simulink model "LLC_simu"  (R2023a)
settings: Solver=VariableStepAuto  StartTime=0.0  StopTime=0.01  RelTol=1e-3
values from neighbouring files (symbols this model uses):
  Co = Co_s    [generate_agent_v2_cases.m]    (also in generate_aging_trajectory.m = co_ratio * Co_nominal; generate_dataset_2.m = co_samples; llc_agent_v2_cases.mat = [0.002046 0.00231 0.001936 0.00209 0.00198 0.002288 0.001892; llc_aging_trajectory.mat = [0.0022 0.002145 0.00209 0.002035 0.00198 0.001925 0.00187 0)
  Cr = Cr_s    [generate_agent_v2_cases.m]    (also in generate_aging_trajectory.m = Cr_nominal * ones(num_sequences, 1); generate_dataset_2.m = cr_samples; llc_agent_v2_cases.mat = [3.57e-08 3.36e-08 3.465e-08 4.55e-08 3.43e-08 3.605e-08 3.5; llc_aging_trajectory.mat = [3.5e-08 3.5e-08 3.5e-08 3.5e-08 3.5e-08 3.5e-08 3.5e-08 3.5)
  D = 45    [generate_agent_v2_cases.m]    (also in generate_aging_trajectory.m; generate_dataset_2.m; setparams.m)
  Lm = Lm_s    [generate_agent_v2_cases.m]    (also in generate_aging_trajectory.m = Lm_nominal * ones(num_sequences, 1); generate_dataset_2.m = lm_samples; llc_agent_v2_cases.mat = [0.00014162 0.0001022 0.00015184 0.00014892 0.00015038 0.000; llc_aging_trajectory.mat = [0.000146 0.000146 0.000146 0.000146 0.000146 0.000146 0.000)
  Lr = Lr_s    [generate_agent_v2_cases.m]    (also in generate_aging_trajectory.m = Lr_nominal * ones(num_sequences, 1); generate_dataset_2.m = lr_samples; llc_agent_v2_cases.mat = [9.49e-05 7.154e-05 7.519e-05 7.081e-05 7.446e-05 7.008e-05 ; llc_aging_trajectory.mat = [7.3e-05 7.3e-05 7.3e-05 7.3e-05 7.3e-05 7.3e-05 7.3e-05 7.3)
  Ro = rload_samples(k)    [generate_aging_trajectory.m]    (also in generate_dataset_2.m; setparams.m = 2)
  T = 1 / fs_k    [generate_agent_v2_cases.m]    (also in generate_aging_trajectory.m = 1.11111111111e-05; generate_dataset_2.m; setparams.m = 1.11111111111e-05)
  Vin = Vin_nominal    (= 311)    [generate_aging_trajectory.m]    (also in generate_dataset_2.m = vin_samples(k); setparams.m)
  Vpulse = 1    [generate_agent_v2_cases.m]    (also in generate_aging_trajectory.m; generate_dataset_2.m; setparams.m)
libraries: spsCurrentMeasurementLib x14, spsSeriesRLCBranchLib x5, spsVoltageMeasurementLib x5, spsDiodeLib x4, spsMosfetLib x4, spsLinearTransformerLib x1, spsDCVoltageSourceLib x1, spspowerguiLib x1
settings Model: Creator=22431  LastModifiedBy=22431
settings SimscapeCC: SimscapeNormalizeSystem=off

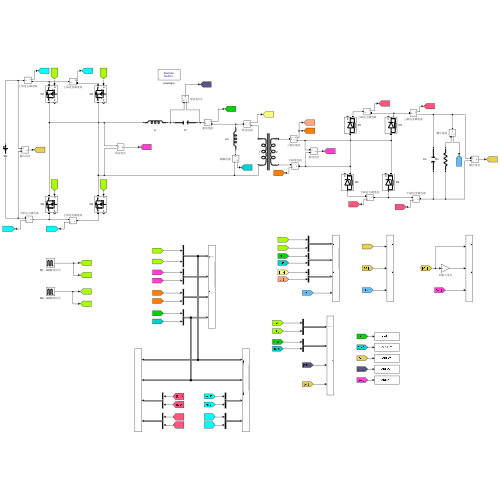
[thumbnail: Simulink's stored preview of the top-level diagram]
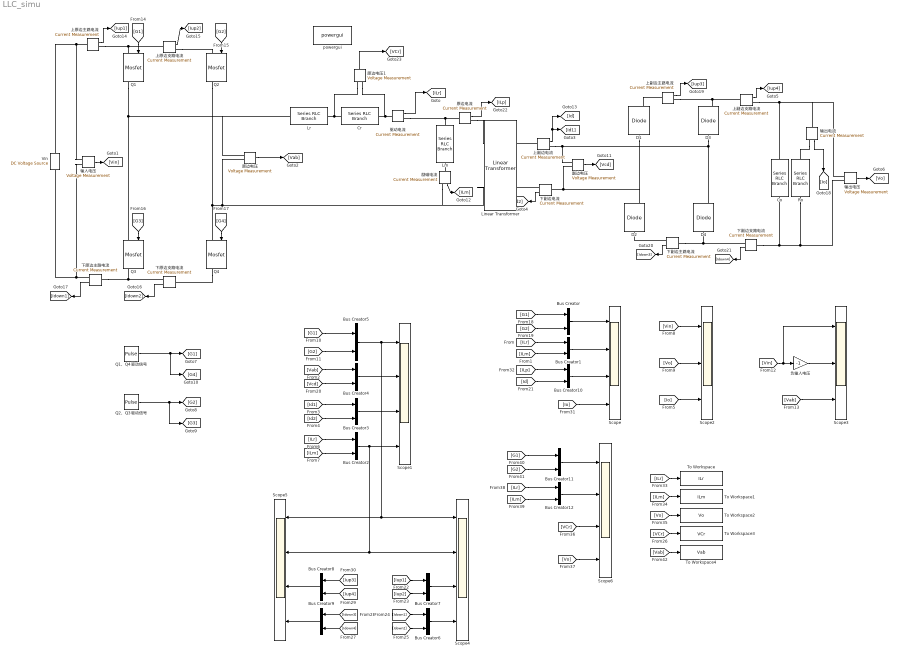
== system LLC_simu ==
  Bus Creator{,1..12} (13 alike) : BusCreator  Inputs=2
  Co : spsSeriesRLCBranchLib/Series RLC Branch  LConnTagsString=__new0  RConnTagsString=__new0  BranchType=C  Resistance=1  Inductance=1e-3  SetiL0=off  InitialCurrent=0  Capacitance=Co  Setx0=off  InitialVoltage=0  Measurements=None
  Cr : spsSeriesRLCBranchLib/Series RLC Branch  LConnTagsString=__new0  RConnTagsString=__new0  BranchType=C  Resistance=1  Inductance=1e-3  SetiL0=off  InitialCurrent=0  Capacitance=Cr  Setx0=off  InitialVoltage=0  Measurements=None
  D{1..4} (4 alike) : spsDiodeLib/Diode  Ron=0.001  Lon=0  Vf=0.8  IC=0  UseSnubber=0  Rs=500  Cs=250e-9  Measurements=on
  Linear Transformer : spsLinearTransformerLib/Linear Transformer  UNITS=SI  NominalPower=[ 250e6 100e3 ]  winding1=[6.5 0 0]  winding2=[1 0 0]  ThreeWindings=off  winding3=[1.5e+05 0 0]  RmLm=[1e6 inf]  Measurements=None  DataType=on
  Lm : spsSeriesRLCBranchLib/Series RLC Branch  LConnTagsString=__new0  RConnTagsString=__new0  BranchType=L  Resistance=1  Inductance=Lm  SetiL0=off  InitialCurrent=0  Capacitance=1e-6  Setx0=off  InitialVoltage=0  Measurements=None
  Lr : spsSeriesRLCBranchLib/Series RLC Branch  LConnTagsString=__new0  RConnTagsString=__new0  BranchType=L  Resistance=1  Inductance=Lr  SetiL0=off  InitialCurrent=0  Capacitance=1e-6  Setx0=off  InitialVoltage=0  Measurements=None
  Q{1..4} (4 alike) : spsMosfetLib/Mosfet  Ron=0.1  Lon=0  Rd=0.01  Vfd=0  IC=0  Rs=1e5  Cs=inf  Measurements=on
  Q1、Q4驱动信号 : DiscretePulseGenerator  PulseType=Time based  Amplitude=Vpulse  Period=T  PulseWidth=D
  Q2、Q3驱动信号 : DiscretePulseGenerator  PulseType=Time based  Amplitude=Vpulse  Period=T  PulseWidth=D  PhaseDelay=T/2
  Ro : spsSeriesRLCBranchLib/Series RLC Branch  LConnTagsString=__new0  RConnTagsString=__new0  BranchType=R  Resistance=Ro  Inductance=1e-3  SetiL0=off  InitialCurrent=0  Capacitance=1e-6  Setx0=off  InitialVoltage=0  Measurements=None
  Scope{,1,4..6} (5 alike) : Scope  NumInputPorts=4
  Scope2 : Scope  NumInputPorts=3
  Scope3 : Scope  NumInputPorts=3
  To Workspace : ToWorkspace  VariableName=ILr  SaveFormat=Timeseries  SampleTime=-1
  To Workspace1 : ToWorkspace  VariableName=ILm  SaveFormat=Timeseries  SampleTime=-1
  To Workspace2 : ToWorkspace  VariableName=Vo  SaveFormat=Timeseries  SampleTime=-1
  To Workspace3 : ToWorkspace  VariableName=VCr  SaveFormat=Timeseries  SampleTime=-1
  To Workspace4 : ToWorkspace  VariableName=Vab  SaveFormat=Timeseries  SampleTime=-1
  Vin : spsDCVoltageSourceLib/DC Voltage Source  Amplitude=Vin  Measurements=None
  powergui : spspowerguiLib/powergui  Priority=1  SimulationMode=Discrete  SampleTime=50e-10  frequency=60  Iterations=50  frequencyindice=0  Pbase=100e6  ErrMax=1e-4  UnitsV=kV  UnitsW=MW  buscounter=0  FunctionMessages=off  echomessages=off  EnableUseOfTLC=off  CurrentSourceSwitches=off  DisableSnubberDevices=off  DisableRonSwitches=off  DisableVfSwitches=off  DisplayEquations=off  AutomaticDiscreteSolvers=off  SolverType=Tustin/Backward Euler (TBE)  Interpol=off  ExternalGateDelay=off  methode=off  Ts=100  x0status=blocks  SPID=on  SwTol=0  HookPort=off  NonlinearTolerance=1e-4  nMaxIteration=100  ContinueOnMaxIteration=off  RestoreLinks=warning  ResistiveCurrentMeasurement=off  Frange=[0:2:500]  Ylog=off  Xlog=on  ShowGrid=off  save=off  variable=ZData  structure=0  ZoomFFT=off  StartTime=0.0  cycles=1  DisplayStyle=1  fundamental=60  FreqAxis=off  MaxFrequency=1000  frequencyindicesteady=1  RmsSteady=1  display=off
  上副边主路电流 : spsCurrentMeasurementLib/Current Measurement  PhasorSimulation=off  OutputType=Complex  PSBequivalent=0
  上副边支路电流 : spsCurrentMeasurementLib/Current Measurement  PhasorSimulation=off  OutputType=Complex  PSBequivalent=0
  上副边电流 : spsCurrentMeasurementLib/Current Measurement  PhasorSimulation=off  OutputType=Complex  PSBequivalent=0
  上原边主路电流 : spsCurrentMeasurementLib/Current Measurement  PhasorSimulation=off  OutputType=Complex  PSBequivalent=0
  上原边支路电流 : spsCurrentMeasurementLib/Current Measurement  PhasorSimulation=off  OutputType=Complex  PSBequivalent=0
  下副边主路电流 : spsCurrentMeasurementLib/Current Measurement  PhasorSimulation=off  OutputType=Complex  PSBequivalent=0
  下副边支路电流 : spsCurrentMeasurementLib/Current Measurement  PhasorSimulation=off  OutputType=Complex  PSBequivalent=0
  下副边电流 : spsCurrentMeasurementLib/Current Measurement  PhasorSimulation=off  OutputType=Complex  PSBequivalent=0
  下原边主路电流 : spsCurrentMeasurementLib/Current Measurement  PhasorSimulation=off  OutputType=Complex  PSBequivalent=0
  下原边支路电流 : spsCurrentMeasurementLib/Current Measurement  PhasorSimulation=off  OutputType=Complex  PSBequivalent=0
  副边电压 : spsVoltageMeasurementLib/Voltage Measurement  PhasorSimulation=off  OutputType=Complex  PSBequivalent=0
  励磁电流 : spsCurrentMeasurementLib/Current Measurement  PhasorSimulation=off  OutputType=Complex  PSBequivalent=0
  原边电压 : spsVoltageMeasurementLib/Voltage Measurement  PhasorSimulation=off  OutputType=Complex  PSBequivalent=0
  原边电压1 : spsVoltageMeasurementLib/Voltage Measurement  PhasorSimulation=off  OutputType=Complex  PSBequivalent=0
  原边电流 : spsCurrentMeasurementLib/Current Measurement  PhasorSimulation=off  OutputType=Complex  PSBequivalent=0
  负输入电压 : Gain  Gain=-1
  输入电压 : spsVoltageMeasurementLib/Voltage Measurement  PhasorSimulation=off  OutputType=Complex  PSBequivalent=0
  输出电压 : spsVoltageMeasurementLib/Voltage Measurement  PhasorSimulation=off  OutputType=Complex  PSBequivalent=0
  输出电流 : spsCurrentMeasurementLib/Current Measurement  PhasorSimulation=off  OutputType=Complex  PSBequivalent=0
  驱动电流 : spsCurrentMeasurementLib/Current Measurement  PhasorSimulation=off  OutputType=Complex  PSBequivalent=0
  wires:
  Bus Creator1/1 -> Scope/2
  Bus Creator/1 -> Scope/1
  驱动电流/1 -> [ILr]
  [ILr] -> Bus Creator1/1
  原边电压/1 -> [Vab]
  上副边支路电流/1 -> [Iup4]
  输出电压/1 -> [Vo]
  [ILr] -> Bus Creator2/1
  Bus Creator2/1 -> Scope5/2, Scope4/2, Scope1/4
  Bus Creator3/1 -> Scope1/3
  [Id2] -> Bus Creator3/2
  [Id1] -> Bus Creator3/1
  输入电压/1 -> [Vin]
  [G1] -> Bus Creator5/1
  [G2] -> Bus Creator5/2
  Bus Creator5/1 -> Scope5/1, Scope4/1, Scope1/1
  Q1、Q4驱动信号/1 -> [G4], [G1]
  Q2、Q3驱动信号/1 -> [G3], [G2]
  [G1] -> Q1/1
  [G2] -> Q2/1
  [G3] -> Q3/1
  [G4] -> Q4/1
  [Io] -> Scope2/3
  [Vo] -> Scope2/2
  [Vin] -> Scope2/1
  [G1] -> Bus Creator/1
  [G2] -> Bus Creator/2
  副边电压/1 -> [Vcd]
  Bus Creator4/1 -> Scope1/2
  [Vcd] -> Bus Creator4/2
  [Vab] -> Bus Creator4/1
  励磁电流/1 -> [ILm]
  [ILm] -> Bus Creator2/2
  [Vab] -> Scope3/3
  负输入电压/1 -> Scope3/2
  [Vin] -> Scope3/1, 负输入电压/1
  上原边主路电流/1 -> [Iup1]
  上原边支路电流/1 -> [Iup2]
  下原边支路电流/1 -> [Idown2]
  下原边主路电流/1 -> [Idown1]
  Bus Creator6/1 -> Scope4/4
  Bus Creator7/1 -> Scope4/3
  [Idown2] -> Bus Creator6/2
  [Idown1] -> Bus Creator6/1
  [Iup2] -> Bus Creator7/2
  [Iup1] -> Bus Creator7/1
  [ILm] -> Bus Creator1/2
  [Io] -> Scope/4
  上副边电流/1 -> [Id1], [Id]
  下副边电流/1 -> [Id2]
  输出电流/1 -> [Io]
  上副边主路电流/1 -> [Iup3]
  下副边主路电流/1 -> [Idown3]
  下副边支路电流/1 -> [Idown4]
  [Idown3] -> Bus Creator9/1
  [Idown4] -> Bus Creator9/2
  [Iup4] -> Bus Creator8/2
  [Iup3] -> Bus Creator8/1
  Bus Creator8/1 -> Scope5/3
  Bus Creator9/1 -> Scope5/4
  原边电流/1 -> [ILp]
  Bus Creator10/1 -> Scope/3
  [ILp] -> Bus Creator10/1
  [Id] -> Bus Creator10/2
  原边电压1/1 -> [VCr]
  [ILr] -> To Workspace/1
  [ILm] -> To Workspace1/1
  [VCr] -> To Workspace3/1
  [Vo] -> To Workspace2/1
  Bus Creator12/1 -> Scope6/2
  [G1] -> Bus Creator11/1
  [G2] -> Bus Creator11/2
  [ILr] -> Bus Creator12/1
  [ILm] -> Bus Creator12/2
  Bus Creator11/1 -> Scope6/1
  [Vab] -> To Workspace4/1
  [VCr] -> Scope6/3
  [Vo] -> Scope6/4
  connections:
  上原边主路电流/RConn1 -- 上原边支路电流/LConn1 -- Q1/LConn1
  输入电压/LConn2 -- 下原边主路电流/RConn1 -- Vin/LConn1
  Q1/RConn1 -- 原边电压/LConn1 -- Lr/LConn1 -- Q3/LConn1
  Q2/RConn1 -- 励磁电流/RConn1 -- Linear Transformer/LConn2 -- 原边电压/LConn2 -- Q4/LConn1
  Cr/LConn1 -- 原边电压1/LConn1 -- Lr/RConn1
  驱动电流/RConn1 -- 原边电流/LConn1 -- Lm/LConn1
  输出电压/LConn2 -- Ro/RConn1 -- Co/RConn1 -- 下副边支路电流/LConn1
  驱动电流/LConn1 -- 原边电压1/LConn2 -- Cr/RConn1
  励磁电流/LConn1 -- Lm/RConn1
  上副边电流/LConn1 -- Linear Transformer/RConn1
  上副边支路电流/RConn1 -- 输出电流/LConn1 -- 输出电压/LConn1 -- Co/LConn1
  输入电压/LConn1 -- 上原边主路电流/LConn1 -- Vin/RConn1
  上原边支路电流/RConn1 -- Q2/LConn1
  Q4/RConn1 -- 下原边支路电流/LConn1
  下原边支路电流/RConn1 -- 下原边主路电流/LConn1 -- Q3/RConn1
  上副边支路电流/LConn1 -- 上副边主路电流/RConn1 -- D3/RConn1
  副边电压/LConn2 -- D1/LConn1 -- D2/RConn1 -- 下副边电流/LConn1
  下副边电流/RConn1 -- Linear Transformer/RConn2
  上副边电流/RConn1 -- D4/RConn1 -- D3/LConn1 -- 副边电压/LConn1
  输出电流/RConn1 -- Ro/LConn1
  上副边主路电流/LConn1 -- D1/RConn1
  下副边支路电流/RConn1 -- 下副边主路电流/LConn1 -- D4/LConn1
  下副边主路电流/RConn1 -- D2/LConn1
  原边电流/RConn1 -- Linear Transformer/LConn1
